simulink model "quadcopter_control"  (R2025b)
settings: Solver=ode45  StartTime=0.0  StopTime=p.stopTime  MaxStep=p.sampleTime  RelTol=1e-8  AbsTol=1e-10
model workspace (MAT data in the model file):
  inputSignal = [0 0.002 0.004 0.006 0.008 0.01 0.012 0.014 0.016 0.018 0.02 0.022 ... (43282 elements, 2546x17)]
  p.mass = 1.2
  p.gravity = 9.81
  p.inertia = [0.012; 0.014; 0.023]
  p.arm = 0.23
  p.thrustCoefficient = 1.1e-05
  p.dragCoefficient = 1.8e-07
  p.rotorTimeConstant = 0.025
  p.maximumRotorSpeed = 900
  p.linearDrag = 0.15
  p.mixer = [1.1e-05  1.1e-05  1.1e-05  1.1e-05; 1.7889801564e-06  1.7889801564e-06  -1.7889801564e-06  -1.7889801564e-06; -1.7889801564e-06  1.7889801564e-06  1.7889801564e-06  -1.7889801564e-06; 1.8e-07  -1.8e-07  1.8e-07  -1.8e-07]
  p.hoverSpeed = 517.247962341
  p.positionKp = [6.25; 6.25; 12]
  p.positionKd = [5; 5; 6]
  p.altitudeKi = 8
  p.angleGain = 8
  p.rateKp = 30
  p.rateKi = 120
  p.rateTracking = 15
  p.altitudeTracking = 4
  p.goal = [1; 0.5; 1.5]
  p.yawGoal = 0.349065850399
  p.tiltLimit = 0.35
  p.takeoffTime = 0.1
  p.takeoffDuration = 1
  p.moveTime = 1.41
  p.moveDuration = 1.2
  p.gustTime = 3.882
  p.gustDuration = 0.2
  p.gustForce = [0.8; -0.5; 0.4]
  p.gustMoment = [0.02; -0.01; 0.005]
  p.sampleTime = 0.002
  p.sizingDuration = 12
  p.stopTime = 5.078
  p.initialState = [0; 0; 0; 0; 0; 0; 0; 0; 0; 0; 0; 0; 517.247962341; 517.247962341; 517.247962341; 517.247962341]
  p.initialControlState = [0; 0; 0; 0]
  p.modelName = 'quadcopter_control'
values from neighbouring files (symbols this model uses):
  p = project_parameters();[p,timing]=plan_experiment(p);[t,state,control,error]=run_simulation(p)    [run_demo.m]
undefined symbols (not defined in the file or in its folder): sl_controller, sl_plant
settings Model: Creator=LENOVO  LastModifiedBy=LENOVO

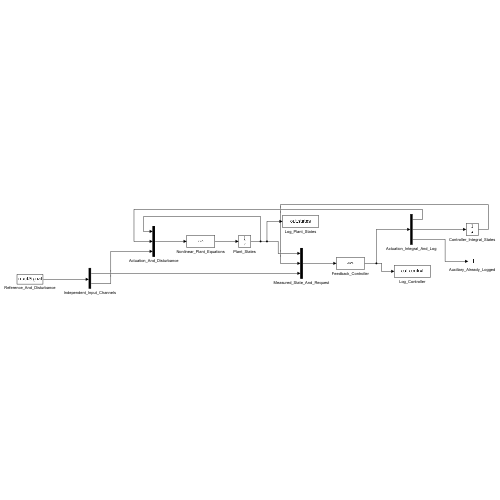
[thumbnail: Simulink's stored preview of the top-level diagram]
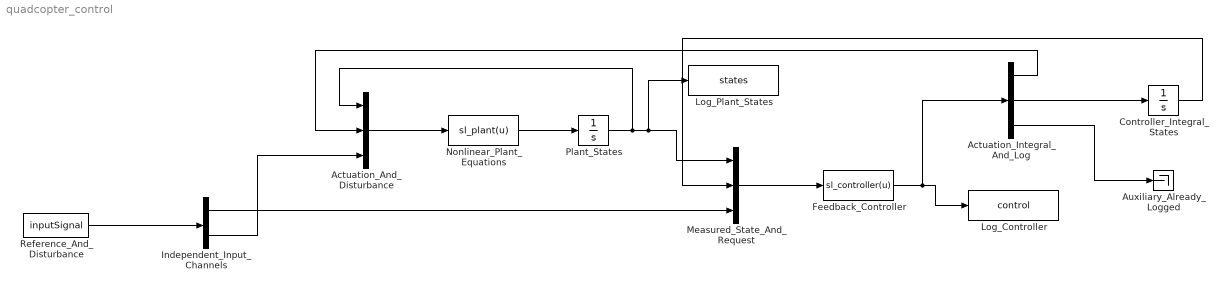
== system quadcopter_control ==
  Actuation_And_Disturbance : Mux  Inputs=3
  Actuation_Integral_And_Log : Demux  Outputs=[4 4 4]
  Auxiliary_Already_Logged : Terminator
  Controller_Integral_States : Integrator  InitialCondition=p.initialControlState
  Feedback_Controller : MATLABFcn  MATLABFcn=sl_controller(u)  OutputDimensions=12
  Independent_Input_Channels : Demux  Outputs=[10 6]
  Log_Controller : ToWorkspace  VariableName=control  SaveFormat=Timeseries  SampleTime=-1
  Log_Plant_States : ToWorkspace  VariableName=states  SaveFormat=Timeseries  SampleTime=-1
  Measured_State_And_Request : Mux  Inputs=3
  Nonlinear_Plant_Equations : MATLABFcn  MATLABFcn=sl_plant(u)  OutputDimensions=16
  Plant_States : Integrator  InitialCondition=p.initialState
  Reference_And_Disturbance : FromWorkspace  VariableName=inputSignal  OutputAfterFinalValue=Holding final value
  wires:
  Nonlinear_Plant_Equations/1 -> Plant_States/1
  Actuation_And_Disturbance/1 -> Nonlinear_Plant_Equations/1
  Independent_Input_Channels/2 -> Actuation_And_Disturbance/3
  Actuation_Integral_And_Log/1 -> Actuation_And_Disturbance/2
  Actuation_Integral_And_Log/3 -> Auxiliary_Already_Logged/1
  Actuation_Integral_And_Log/2 -> Controller_Integral_States/1
  Feedback_Controller/1 -> Actuation_Integral_And_Log/1, Log_Controller/1
  Measured_State_And_Request/1 -> Feedback_Controller/1
  Independent_Input_Channels/1 -> Measured_State_And_Request/3
  Controller_Integral_States/1 -> Measured_State_And_Request/2
  Plant_States/1 -> Measured_State_And_Request/1, Log_Plant_States/1, Actuation_And_Disturbance/1
  Reference_And_Disturbance/1 -> Independent_Input_Channels/1
